simulink library "Yaw_Ideal_Actuator_Lib"  (R2025a)
settings: Solver=ode45  StartTime=0.0  StopTime=10.0  RelTol=1e-3  EnableMultiTasking=on
undefined symbols (not defined in the file): WT_Params
Description:
  | Copyright 2009-2025 The MathWorks, Inc. MathWorks, Inc.
settings Model: Creator=smiller  LastModifiedBy=smiller
settings SolverCC: AlgebraicLoopSolver=TrustRegion
settings DataIOCC: LimitDataPoints=on  SaveFormat=Array  SignalLoggingSaveFormat=ModelDataLogs  ReturnWorkspaceOutputs=off
settings OptimizationCC: ReuseModelBlockBuffer=off  ExpressionDepthLimit=2147483647.0  LifeSpan=inf
settings DebuggingCC: UnderspecifiedInitializationDetection=Classic  MergeDetectMultiDrivingBlocksExec=none  SolverPrmCheckMsg=warning  FcnCallInpInsideContextMsg=warning  UnconnectedInputMsg=warning  UnconnectedOutputMsg=warning  UnconnectedLineMsg=warning  AllowSymbolicDim=off  StateNameClashWarn=warning  PregeneratedLibrarySubsystemCodeDiagnostic=none  SFUnexpectedBacktrackingDiag=warning  SFNoUnconditionalDefaultTransitionDiag=warning  SFExecutionAtInitializationDiag=none  ArithmeticOperatorsInVariantConditions=warning
settings HardwareCC: ProdBitPerPointer=32.0  ProdBitPerSizeT=32.0  ProdBitPerPtrDiffT=32.0  ProdLargestAtomicFloat=None  ProdIntDivRoundTo=Undefined  ProdEndianess=Unspecified  ProdWordSize=32.0  ProdHWDeviceType=32-bit Generic
settings ModelReferenceCC: EnableRefExpFcnMdlSchedulingChecks=on  PropagateSignalLabelsOutOfModel=off
settings SFSimCC: SimUseLocalCustomCode=off  CustomCodeUndefinedFunction=UseInterfaceOnly
settings RTWCC: RTWUseLocalCustomCode=off  GPUComputeCapability=3.5  DLArmComputeVersion=19.05
settings CodeAppCC: StateflowObjectComments=on
settings GRTTargetCC: TargetLangStandard=C89/C90 (ANSI)  CombineOutputUpdateFcns=off  GRTInterface=on
settings ConfigComp: CovMetricSettings=dw  CovSaveCumulativeToWorkspaceVar=on  CovSaveSingleToWorkspaceVar=on  CovExternalEMLEnable=off  CovSFcnEnable=off

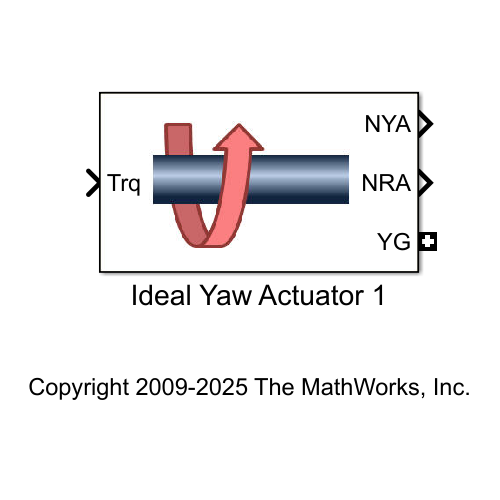
[thumbnail: Simulink's stored preview of the top-level diagram]
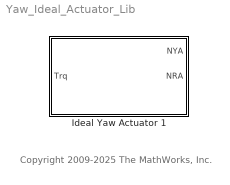
== system Yaw_Ideal_Actuator_Lib ==
  note: Copyright 2009-2025 The MathWorks, Inc.
  Ideal Yaw Actuator 1 : Subsystem
      mask Display: image('Yaw_Ideal_Actuator_Horizontal_IMAGE.jpg');

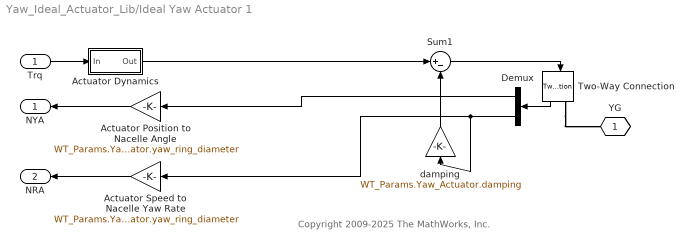
== system Yaw_Ideal_Actuator_Lib/Ideal Yaw Actuator 1 ==
  note: Copyright 2009-2025 The MathWorks, Inc.
  Trq : Inport
  Actuator Dynamics : Subsystem  mask(First-order lag supporting vector signals){b=WT_Params.Yaw_Actuator.ideal_actuator_time_constant, x_initial=0}
      mask prompts: b "Filter time constant"; x_initial "Initial output"
      mask help: Models a lag of the form 1/(b*s+1) where s is the Laplace operator.
  Actuator Position to Nacelle Angle : Gain  Gain=WT_Params.Yaw_Actuator.yaw_gear_diameter/WT_Params.Yaw_Actuator.yaw_ring_diameter
  Actuator Speed to Nacelle Yaw Rate : Gain  Gain=WT_Params.Yaw_Actuator.yaw_gear_diameter/WT_Params.Yaw_Actuator.yaw_ring_diameter
  Demux : Demux  Outputs=2
  Sum1 : Sum  Inputs=|+-
  Two-Way Connection : TwoWayConnection
  damping : Gain  Gain=WT_Params.Yaw_Actuator.damping
  YG : PMIOPort  Tag=PMCPort  Side=Right
  NYA : Outport  VectorParamsAs1DForOutWhenUnconnected=off
  NRA : Outport  Port=2  VectorParamsAs1DForOutWhenUnconnected=off
  wires:
  damping/1 -> Sum1/2
  Demux/2 -> damping/1, Actuator Speed to Nacelle Yaw Rate/1
  Demux/1 -> Actuator Position to Nacelle Angle/1
  Actuator Position to Nacelle Angle/1 -> NYA/1
  Actuator Speed to Nacelle Yaw Rate/1 -> NRA/1
  Trq/1 -> Actuator Dynamics/1(In)
  Actuator Dynamics/1(Out) -> Sum1/1
  Sum1/1 -> Two-Way Connection/1
  Two-Way Connection/1 -> Demux/1
  connections:
  Two-Way Connection/RConn1 -- YG/RConn1

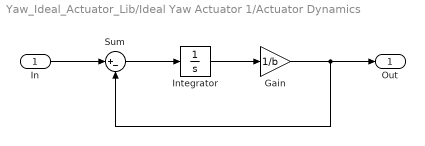
== system Yaw_Ideal_Actuator_Lib/Ideal Yaw Actuator 1/Actuator Dynamics ==
  In : Inport
  Gain : Gain  Gain=1/b
  Integrator : Integrator  InitialCondition=x_initial
  Sum : Sum  Inputs=|+-  InputSameDT=on  SaturateOnIntegerOverflow=on  OutDataTypeStr=Inherit: Same as first input
  Out : Outport  VectorParamsAs1DForOutWhenUnconnected=off
  wires:
  Sum/1 -> Integrator/1
  In/1 -> Sum/1
  Integrator/1 -> Gain/1
  Gain/1 -> Sum/2, Out/1
